simulink model "Deadbeat_discrete"  (R2018b)
settings: Solver=VariableStepAuto  StartTime=0.0  StopTime=100  RelTol=1e-3
libraries: simulink x1
settings Model: Creator=giuli  LastModifiedBy=gimih
settings SFSimCC: SimUseLocalCustomCode=off
settings RTWCC: RTWUseLocalCustomCode=off

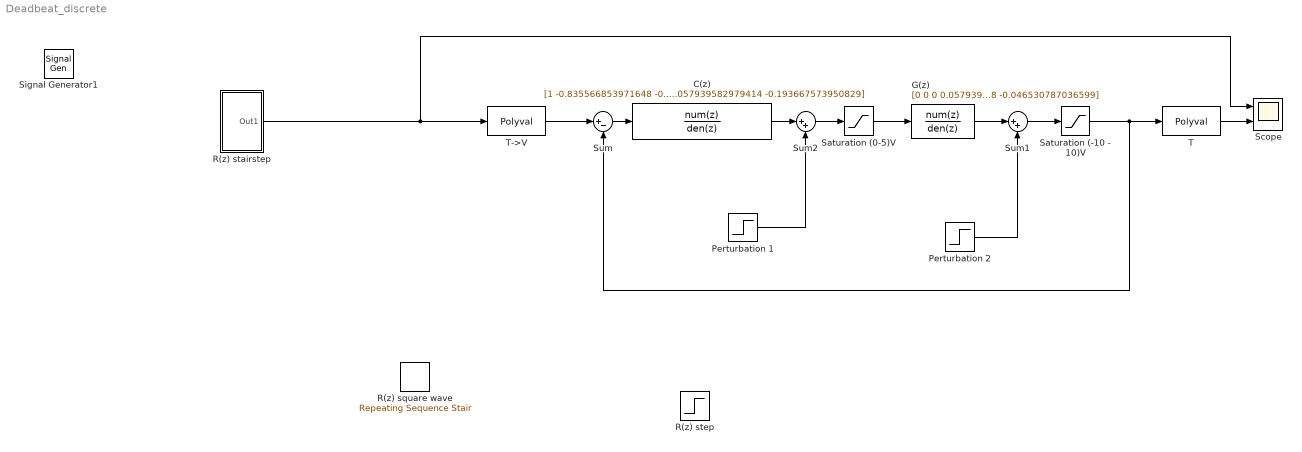
== system Deadbeat_discrete ==
  C(z) : DiscreteFilter  Numerator=[1 -0.835566853971648 -0.046530787036599]  Denominator=[6291/25000 0 0 -0.057939582979414 -0.193667573950829]  SampleTime=0.08
  G(z) : DiscreteFilter  Numerator=[0 0 0 0.057939582979414 0.193667573950829]  Denominator=[1 -0.835566853971648 -0.046530787036599]  SampleTime=0.08
  Perturbation 1 : Step  Time=20  After=5  SampleTime=0
  Perturbation 2 : Step  Time=35  After=-5  SampleTime=0
  R(z) square wave : simulink/Sources/Repeating Sequence Stair  OutValues=[30 45 40 50 35 30 50].'  tsamp=5  OutMin=[]  OutMax=[]  OutDataTypeStr=double  OutputDataTypeScalingMode=double  OutDataType=fixdt(0,8)  ConRadixGroup=Best Precision: Vector-wise  OutScaling=2^-12
  R(z) stairstep : Subsystem
  "R(z) step " : Step  Time=30  Before=30  After=50  SampleTime=0.08
  Saturation (-10 - 10)V : Saturate  UpperLimit=10  LowerLimit=-10
  Saturation (0-5)V : Saturate  UpperLimit=5  LowerLimit=0
  Scope : Scope  NumInputPorts=2
  Signal Generator1 : SignalGenerator  WaveForm=random  Amplitude=10  Frequency=0.01
  Sum : Sum  Inputs=|+-
  Sum1 : Sum  Inputs=|++
  Sum2 : Sum  Inputs=|++
  T : Polyval  Coefs=[2.865 26.323]
  T->V : Polyval  Coefs=[1/2.865 -26.323/2.865]
  wires:
  Saturation (-10 - 10)V/1 -> T/1, Sum/2
  T->V/1 -> Sum/1
  T/1 -> Scope/2
  Saturation (0-5)V/1 -> G(z)/1
  Sum/1 -> C(z)/1
  R(z) stairstep/1(Out1) -> T->V/1, Scope/1
  C(z)/1 -> Sum2/1
  Sum2/1 -> Saturation (0-5)V/1
  G(z)/1 -> Sum1/1
  Sum1/1 -> Saturation (-10 - 10)V/1
  Perturbation 1/1 -> Sum2/2
  Perturbation 2/1 -> Sum1/2

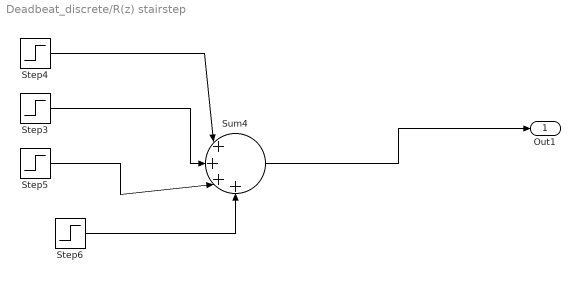
== system Deadbeat_discrete/R(z) stairstep ==
  Step3 : Step  Time=15  Before=30  After=35  SampleTime=0
  Step4 : Step  Time=25  After=5  SampleTime=0
  Step5 : Step  Time=35  After=5  SampleTime=0
  Step6 : Step  Time=45  After=5  SampleTime=0
  Sum4 : Sum  Inputs=|++++
  Out1 : Outport
  wires:
  Step5/1 -> Sum4/3
  Step4/1 -> Sum4/1
  Step6/1 -> Sum4/4
  Step3/1 -> Sum4/2
  Sum4/1 -> Out1/1
